simulink model "attitude_control"  (R2025b)
settings: Solver=ode45  StartTime=0.0  StopTime=600  MaxStep=1  RelTol=1e-11  AbsTol=1e-12
values from neighbouring files (symbols this model uses):
  beta0 = beta0(:)    [run_crosscheck.m]
  omega0 = omega0(:)    [run_crosscheck.m]
undefined symbols (not defined in the file or in its folder): J, K, P, U_MAX
settings Model: Creator=avaza  LastModifiedBy=avaza
settings DataIOCC: SaveOutput=off  SaveTime=off  OutputOption=SpecifiedOutputTimes  OutputTimes=0:0.2:600

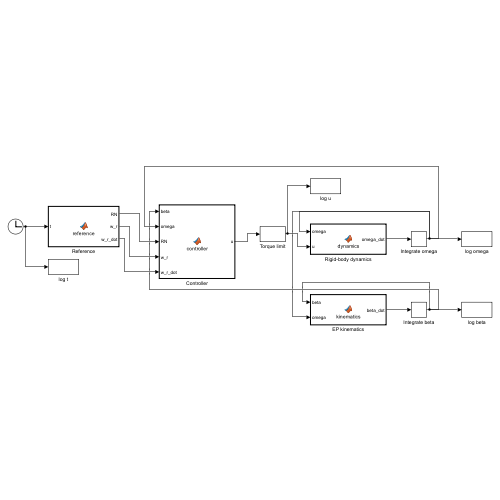
[thumbnail: Simulink's stored preview of the top-level diagram]
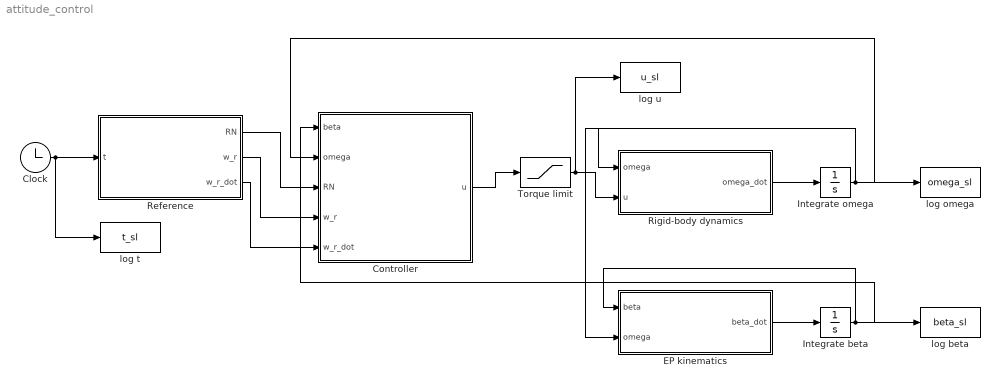
== system attitude_control ==
  Clock : Clock
  Controller : MATLAB Function  TreatAsAtomicUnit=on
  EP kinematics : MATLAB Function  TreatAsAtomicUnit=on
  Integrate beta : Integrator  InitialCondition=beta0(:)
  Integrate omega : Integrator  InitialCondition=omega0(:)
  Reference : MATLAB Function  TreatAsAtomicUnit=on
  Rigid-body dynamics : MATLAB Function  TreatAsAtomicUnit=on
  Torque limit : Saturate  UpperLimit=U_MAX  LowerLimit=-U_MAX
  log beta : ToWorkspace  VariableName=beta_sl  SampleTime=-1
  log omega : ToWorkspace  VariableName=omega_sl  SampleTime=-1
  log t : ToWorkspace  VariableName=t_sl  SampleTime=-1
  log u : ToWorkspace  VariableName=u_sl  SampleTime=-1
  wires:
  Clock/1 -> Reference/1(t), log t/1
  Reference/1(RN) -> Controller/3(RN)
  Reference/2(w_r) -> Controller/4(w_r)
  Reference/3(w_r_dot) -> Controller/5(w_r_dot)
  Integrate beta/1 -> Controller/1(beta), EP kinematics/1(beta), log beta/1
  Integrate omega/1 -> Controller/2(omega), Rigid-body dynamics/1(omega), EP kinematics/2(omega), log omega/1
  Controller/1(u) -> Torque limit/1
  Torque limit/1 -> Rigid-body dynamics/2(u), log u/1
  Rigid-body dynamics/1(omega_dot) -> Integrate omega/1
  EP kinematics/1(beta_dot) -> Integrate beta/1

== matlab function attitude_control/Controller ==
  data: beta input; u output; omega input; RN input; w_r input; w_r_dot input; J parameter; K parameter; P parameter
function u = controller(beta, omega, RN, w_r, w_r_dot, J, K, P)
% Lyapunov tracking law (unsaturated; the limit is a separate block)
BN = ep2dcm(beta);
e_b = dcm2ep(BN*RN.');                    % error EPs of B relative to R
w_rB = BN*w_r;
w_rdotB = BN*w_r_dot - cross(omega, w_rB); % derivative seen from B
dw = omega - w_rB;
u = -K*e_b(2:4) - P*dw + J*w_rdotB + cross(omega, J*omega);
end

function C = ep2dcm(b)
C = [b(1)^2+b(2)^2-b(3)^2-b(4)^2, 2*(b(2)*b(3)+b(1)*b(4)), 2*(b(2)*b(4)-b(1)*b(3));
     2*(b(2)*b(3)-b(1)*b(4)), b(1)^2-b(2)^2+b(3)^2-b(4)^2, 2*(b(3)*b(4)+b(1)*b(2));
     2*(b(2)*b(4)+b(1)*b(3)), 2*(b(3)*b(4)-b(1)*b(2)), b(1)^2-b(2)^2-b(3)^2+b(4)^2];
end

function b = dcm2ep(C)
% Sheppard's method, short-rotation set (b0 >= 0)
tr = trace(C);
b2 = [(1+tr)/4; (1+2*C(1,1)-tr)/4; (1+2*C(2,2)-tr)/4; (1+2*C(3,3)-tr)/4];
[~, i] = max(b2);
b = zeros(4,1);
b(i) = sqrt(b2(i));
switch i
  case 1
    b(2) = (C(2,3)-C(3,2))/(4*b(1)); b(3) = (C(3,1)-C(1,3))/(4*b(1)); b(4) = (C(1,2)-C(2,1))/(4*b(1));
  case 2
    b(1) = (C(2,3)-C(3,2))/(4*b(2)); b(3) = (C(1,2)+C(2,1))/(4*b(2)); b(4) = (C(3,1)+C(1,3))/(4*b(2));
  case 3
    b(1) = (C(3,1)-C(1,3))/(4*b(3)); b(2) = (C(1,2)+C(2,1))/(4*b(3)); b(4) = (C(2,3)+C(3,2))/(4*b(3));
  otherwise
    b(1) = (C(1,2)-C(2,1))/(4*b(4)); b(2) = (C(3,1)+C(1,3))/(4*b(4)); b(3) = (C(2,3)+C(3,2))/(4*b(4));
end
if b(1) < 0, b = -b; end
end

== matlab function attitude_control/Reference ==
  data: t input; RN output; w_r output; w_r_dot output; n parameter
function [RN, w_r, w_r_dot] = reference(t, n)
% Reference frame R at the V-bar hold point: r1 = along-track (towards the
% target), r3 = orbit normal. LVLH rotates at n about the orbit normal.
th = n*t;
r1 = [-sin(th); cos(th); 0];
r3 = [0; 0; 1];
r2 = cross(r3, r1);
RN = [r1.'; r2.'; r3.'];
w_r = [0; 0; n];
w_r_dot = [0; 0; 0];

== matlab function attitude_control/Rigid-body dynamics ==
  data: omega input; u input; omega_dot output; J parameter
function omega_dot = dynamics(omega, u, J)
% Euler's rotational equations of motion
omega_dot = J \ (-cross(omega, J*omega) + u);

== matlab function attitude_control/EP kinematics ==
  data: beta input; beta_dot output; omega input
function beta_dot = kinematics(beta, omega)
% Euler-parameter kinematic differential equation
B = [-beta(2) -beta(3) -beta(4);
      beta(1) -beta(4)  beta(3);
      beta(4)  beta(1) -beta(2);
     -beta(3)  beta(2)  beta(1)];
beta_dot = 0.5*B*omega;
